simulink model "H12_JB_PE"  (R2026a)
settings: Solver=VariableStepAuto  StopTime=2  MaxStep=2e-3
InitFcn:
  | % Modellparaméterek
  | B = 5e-4;
  | J = 500e-7;
  | 
  | % Kezdeti érték
  | omega_M0 = 100;
settings Model: Creator=Szalay  LastModifiedBy=Szalay

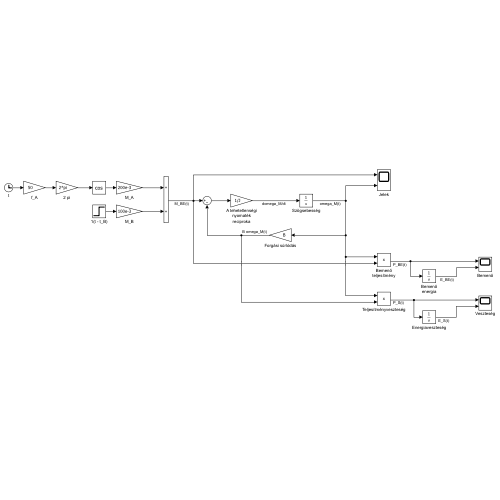
[thumbnail: Simulink's stored preview of the top-level diagram]
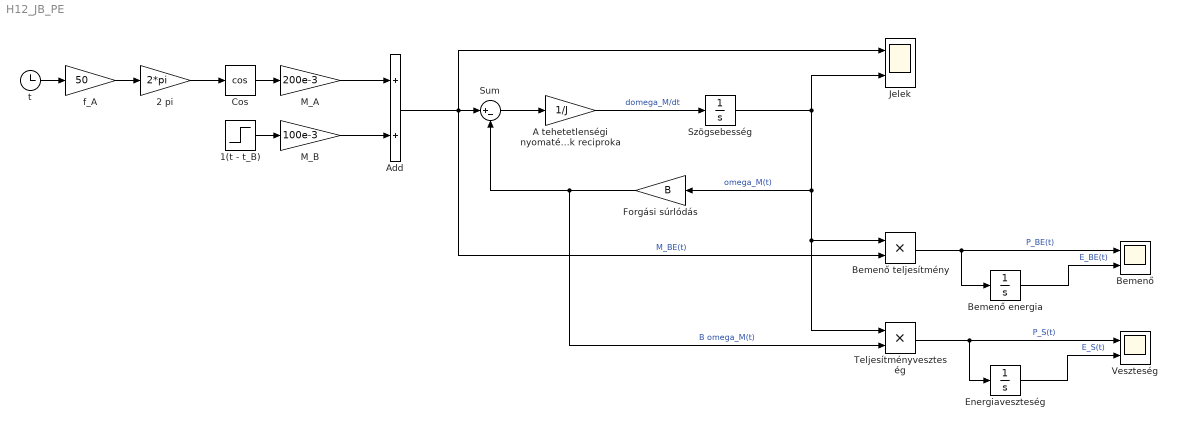
== system H12_JB_PE ==
  1(t - t_B) : Step  Time=1250e-3  SampleTime=0
  2 pi : Gain  Gain=2*pi
  A tehetetlenségi nyomaték reciproka : Gain  Gain=1/J
  Add : Sum
  Bemenő : Scope  NumInputPorts=2
      settings: ActiveDisplayYMinimum=-1.6880057735353147  ActiveDisplayYMaximum=14.720948448174534
  Bemenő energia : Integrator
  Bemenő teljesítmény : Product
  Cos : Trigonometry  Operator=cos
  Energiaveszteség : Integrator
  Forgási súrlódás : Gain  Gain=B
  Jelek : Scope  NumInputPorts=2
      settings: ActiveDisplayYMinimum=-1  ActiveDisplayYMaximum=1
  M_A : Gain  Gain=200e-3
  M_B : Gain  Gain=100e-3
  Sum : Sum  Inputs=|+-
  Szögsebesség : Integrator  InitialCondition=omega_M0
  Teljesítményveszteség : Product
  Veszteség : Scope  NumInputPorts=2
      settings: ActiveDisplayYMinimum=-1.5408886232214034  ActiveDisplayYMaximum=13.867997608992635  DataLoggingVariableName=ScopeData2
  f_A : Gain  Gain=50
  t : Clock
  wires:
  Szögsebesség/1 -> Jelek/2, Teljesítményveszteség/1, Bemenő teljesítmény/1, Forgási súrlódás/1  "omega_M(t)"
  A tehetetlenségi nyomaték reciproka/1 -> Szögsebesség/1  "domega_M/dt"
  Sum/1 -> A tehetetlenségi nyomaték reciproka/1
  Forgási súrlódás/1 -> Teljesítményveszteség/2, Sum/2  "B omega_M(t)"
  Add/1 -> Bemenő teljesítmény/2, Jelek/1, Sum/1  "M_BE(t)"
  M_A/1 -> Add/1
  Cos/1 -> M_A/1
  t/1 -> f_A/1
  f_A/1 -> 2 pi/1
  2 pi/1 -> Cos/1
  M_B/1 -> Add/2
  1(t - t_B)/1 -> M_B/1
  Bemenő teljesítmény/1 -> Bemenő energia/1, Bemenő/1  "P_BE(t)"
  Bemenő energia/1 -> Bemenő/2  "E_BE(t)"
  Teljesítményveszteség/1 -> Veszteség/1, Energiaveszteség/1  "P_S(t)"
  Energiaveszteség/1 -> Veszteség/2  "E_S(t)"
